simulink model "ex1s"  (R2022a)
settings: Solver=VariableStepAuto  StartTime=0.0  StopTime=10  RelTol=1e-3
settings Model: Creator=Guilherme  LastModifiedBy=Guilherme

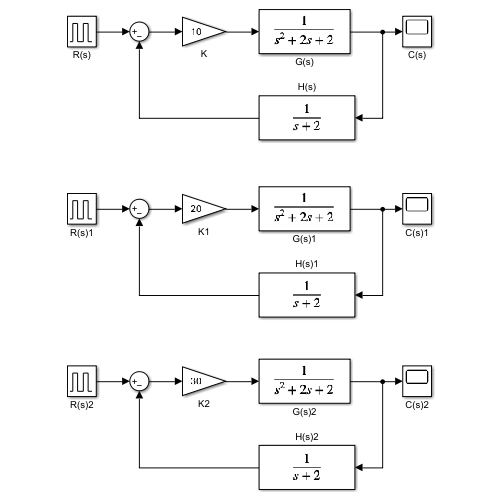
[thumbnail: Simulink's stored preview of the top-level diagram]
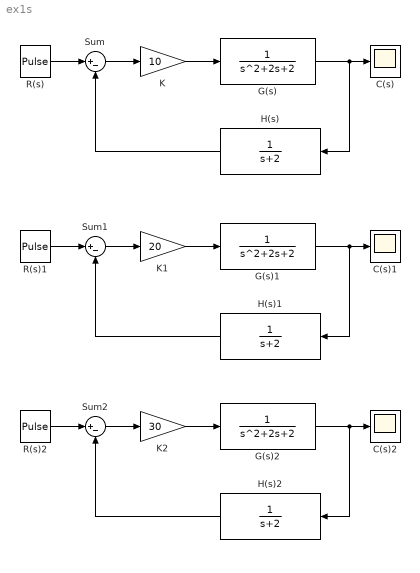
== system ex1s ==
  C(s) : Scope
  C(s)1 : Scope
  C(s)2 : Scope
  G(s) : TransferFcn  Denominator=[1 2 2]
  G(s)1 : TransferFcn  Denominator=[1 2 2]
  G(s)2 : TransferFcn  Denominator=[1 2 2]
  H(s) : TransferFcn  Denominator=[1 2]
  H(s)1 : TransferFcn  Denominator=[1 2]
  H(s)2 : TransferFcn  Denominator=[1 2]
  K : Gain  Gain=10
  K1 : Gain  Gain=20
  K2 : Gain  Gain=30
  R(s) : DiscretePulseGenerator  PulseType=Time based  Amplitude=10  Period=20  PulseWidth=0.5  PhaseDelay=1
  R(s)1 : DiscretePulseGenerator  PulseType=Time based  Amplitude=10  Period=20  PulseWidth=0.5  PhaseDelay=1
  R(s)2 : DiscretePulseGenerator  PulseType=Time based  Amplitude=10  Period=20  PulseWidth=0.5  PhaseDelay=1
  Sum : Sum  Inputs=|+-
  Sum1 : Sum  Inputs=|+-
  Sum2 : Sum  Inputs=|+-
  wires:
  Sum/1 -> K/1
  G(s)/1 -> H(s)/1, C(s)/1
  H(s)/1 -> Sum/2
  R(s)/1 -> Sum/1
  K/1 -> G(s)/1
  H(s)1/1 -> Sum1/2
  G(s)1/1 -> H(s)1/1, C(s)1/1
  Sum1/1 -> K1/1
  K1/1 -> G(s)1/1
  R(s)1/1 -> Sum1/1
  Sum2/1 -> K2/1
  G(s)2/1 -> H(s)2/1, C(s)2/1
  H(s)2/1 -> Sum2/2
  R(s)2/1 -> Sum2/1
  K2/1 -> G(s)2/1
